simulink model "pfb_fft_d3a"  (R2021a)
settings: Solver=VariableStepAuto  StartTime=0.0  StopTime=100.0  RelTol=1e-3
undefined symbols (not defined in the file): i, pfb_coeff_gen_calc
libraries: xbsIndex_r4 x11529, casper_library_misc x39, casper_library_delays x39, xbsReplacements_r4 x2
(part 38 of 118)

== system pfb_fft_d3a/fft_wideband_real/fft_biplex_real_4x/bi_real_unscr_4x/mirror_spectrum/dmux2 ==
  sel : Inport
  d0 : Inport  Port=2
  d1 : Inport  Port=3
  d_bussify : Subsystem  AncestorBlock=casper_library_flow_control/bus_create  mask(bus_create){inputNum=2}
      mask prompts: inputNum "Number of inputs:"
      mask init:
      | bus_create_init(gcb,...
      |     'inputNum', inputNum);
  expand0 : Subsystem  AncestorBlock=casper_library_flow_control/bus_expand  mask(bus_expand){mode=divisions of arbitrary size, outputNum=2, outputWidth=[36 36], outputBinaryPt=[0  0], outputArithmeticType=[0  0], show_format=on, outputToWorkspace=off, variablePrefix=, outputToModelAsWell=on}
      mask prompts: outputNum "Number of outputs:"; outputWidth "Output width:"; outputBinaryPt "Output binary point position:"; outputArithmeticType "Output arithmetic type (ufix=0, fix=1, bool=2):"; show_format "Print format string?"; outputToWorkspace "Output to workspace?"; variablePrefix "Variable name prefix:"; outputToModelAsWell "Output to model as well?"
      mask help:
      | Expands a 'bus' made using a bus_create or Xilinx
      | concat block.
      | The input will be divided into the specified number
      | of outputs with the specified arithmetic types.
      | Divisions are made from most significant bit.
      mask init: same as pfb_fft_d3a/fft_wideband_real/fft_biplex_real_4x/pol0_debus
      settings: AttributesFormatString=2 outputs: uf36.0,uf36.0,
      mask TypeOptions mode: divisions of equal size | divisions of arbitrary size
      mask Callback mode: %bus_expand_callback();
      mask Callback outputWidth: %bus_expand_callback();
      mask Callback outputToWorkspace: %bus_expand_callback();
  expand1 : Subsystem  AncestorBlock=casper_library_flow_control/bus_expand  mask(bus_expand){mode=divisions of arbitrary size, outputNum=2, outputWidth=[36 36], outputBinaryPt=[0  0], outputArithmeticType=[0  0], show_format=on, outputToWorkspace=off, variablePrefix=, outputToModelAsWell=on}
      mask prompts: outputNum "Number of outputs:"; outputWidth "Output width:"; outputBinaryPt "Output binary point position:"; outputArithmeticType "Output arithmetic type (ufix=0, fix=1, bool=2):"; show_format "Print format string?"; outputToWorkspace "Output to workspace?"; variablePrefix "Variable name prefix:"; outputToModelAsWell "Output to model as well?"
      mask help:
      | Expands a 'bus' made using a bus_create or Xilinx
      | concat block.
      | The input will be divided into the specified number
      | of outputs with the specified arithmetic types.
      | Divisions are made from most significant bit.
      mask init: same as pfb_fft_d3a/fft_wideband_real/fft_biplex_real_4x/pol0_debus
      settings: AttributesFormatString=2 outputs: uf36.0,uf36.0,
      mask TypeOptions mode: divisions of equal size | divisions of arbitrary size
      mask Callback mode: %bus_expand_callback();
      mask Callback outputWidth: %bus_expand_callback();
      mask Callback outputToWorkspace: %bus_expand_callback();
  mux0 : xbsIndex_r4/Mux  inputs=2  en=off  latency=1  precision=Full  arith_type=Unsigned  n_bits=16  bin_pt=14  quantization=Truncate  overflow=Wrap  dbl_ovrd=off  block_type=mux
  mux1 : xbsIndex_r4/Mux  inputs=2  en=off  latency=1  precision=Full  arith_type=Unsigned  n_bits=16  bin_pt=14  quantization=Truncate  overflow=Wrap  dbl_ovrd=off  block_type=mux
  sel_expand : Subsystem  AncestorBlock=casper_library_flow_control/bus_expand  mask(bus_expand){mode=divisions of equal size, outputNum=2, outputWidth=1, outputBinaryPt=0, outputArithmeticType=0, show_format=on, outputToWorkspace=off, variablePrefix=, outputToModelAsWell=on}
      mask prompts: outputNum "Number of outputs:"; outputWidth "Output width:"; outputBinaryPt "Output binary point position:"; outputArithmeticType "Output arithmetic type (ufix=0, fix=1, bool=2):"; show_format "Print format string?"; outputToWorkspace "Output to workspace?"; variablePrefix "Variable name prefix:"; outputToModelAsWell "Output to model as well?"
      mask help:
      | Expands a 'bus' made using a bus_create or Xilinx
      | concat block.
      | The input will be divided into the specified number
      | of outputs with the specified arithmetic types.
      | Divisions are made from most significant bit.
      mask init: same as pfb_fft_d3a/fft_wideband_real/fft_biplex_real_4x/pol0_debus
      settings: AttributesFormatString=2 outputs: uf1.0,uf1.0,
      mask TypeOptions mode: divisions of equal size | divisions of arbitrary size
      mask Callback mode: %bus_expand_callback();
      mask Callback outputWidth: %bus_expand_callback();
      mask Callback outputToWorkspace: %bus_expand_callback();
  out : Outport
  wires:
  sel/1 -> sel_expand/1(bus_in)
  d0/1 -> expand0/1(bus_in)
  d1/1 -> expand1/1(bus_in)
  sel_expand/1(msb_out2) -> mux0/1
  expand0/1(msb_out2) -> mux0/2
  expand1/1(msb_out2) -> mux0/3
  sel_expand/2(lsb_out1) -> mux1/1
  expand0/2(lsb_out1) -> mux1/2
  expand1/2(lsb_out1) -> mux1/3
  mux0/1 -> d_bussify/1(in1)
  mux1/1 -> d_bussify/2(in2)
  d_bussify/1(bus_out) -> out/1

== system pfb_fft_d3a/fft_wideband_real/fft_biplex_real_4x/bi_real_unscr_4x/mirror_spectrum/dmux3 ==
  sel : Inport
  d0 : Inport  Port=2
  d1 : Inport  Port=3
  d_bussify : Subsystem  AncestorBlock=casper_library_flow_control/bus_create  mask(bus_create){inputNum=2}
      mask prompts: inputNum "Number of inputs:"
      mask init:
      | bus_create_init(gcb,...
      |     'inputNum', inputNum);
  expand0 : Subsystem  AncestorBlock=casper_library_flow_control/bus_expand  mask(bus_expand){mode=divisions of arbitrary size, outputNum=2, outputWidth=[36 36], outputBinaryPt=[0  0], outputArithmeticType=[0  0], show_format=on, outputToWorkspace=off, variablePrefix=, outputToModelAsWell=on}
      mask prompts: outputNum "Number of outputs:"; outputWidth "Output width:"; outputBinaryPt "Output binary point position:"; outputArithmeticType "Output arithmetic type (ufix=0, fix=1, bool=2):"; show_format "Print format string?"; outputToWorkspace "Output to workspace?"; variablePrefix "Variable name prefix:"; outputToModelAsWell "Output to model as well?"
      mask help:
      | Expands a 'bus' made using a bus_create or Xilinx
      | concat block.
      | The input will be divided into the specified number
      | of outputs with the specified arithmetic types.
      | Divisions are made from most significant bit.
      mask init: same as pfb_fft_d3a/fft_wideband_real/fft_biplex_real_4x/pol0_debus
      settings: AttributesFormatString=2 outputs: uf36.0,uf36.0,
      mask TypeOptions mode: divisions of equal size | divisions of arbitrary size
      mask Callback mode: %bus_expand_callback();
      mask Callback outputWidth: %bus_expand_callback();
      mask Callback outputToWorkspace: %bus_expand_callback();
  expand1 : Subsystem  AncestorBlock=casper_library_flow_control/bus_expand  mask(bus_expand){mode=divisions of arbitrary size, outputNum=2, outputWidth=[36 36], outputBinaryPt=[0  0], outputArithmeticType=[0  0], show_format=on, outputToWorkspace=off, variablePrefix=, outputToModelAsWell=on}
      mask prompts: outputNum "Number of outputs:"; outputWidth "Output width:"; outputBinaryPt "Output binary point position:"; outputArithmeticType "Output arithmetic type (ufix=0, fix=1, bool=2):"; show_format "Print format string?"; outputToWorkspace "Output to workspace?"; variablePrefix "Variable name prefix:"; outputToModelAsWell "Output to model as well?"
      mask help:
      | Expands a 'bus' made using a bus_create or Xilinx
      | concat block.
      | The input will be divided into the specified number
      | of outputs with the specified arithmetic types.
      | Divisions are made from most significant bit.
      mask init: same as pfb_fft_d3a/fft_wideband_real/fft_biplex_real_4x/pol0_debus
      settings: AttributesFormatString=2 outputs: uf36.0,uf36.0,
      mask TypeOptions mode: divisions of equal size | divisions of arbitrary size
      mask Callback mode: %bus_expand_callback();
      mask Callback outputWidth: %bus_expand_callback();
      mask Callback outputToWorkspace: %bus_expand_callback();
  mux0 : xbsIndex_r4/Mux  inputs=2  en=off  latency=1  precision=Full  arith_type=Unsigned  n_bits=16  bin_pt=14  quantization=Truncate  overflow=Wrap  dbl_ovrd=off  block_type=mux
  mux1 : xbsIndex_r4/Mux  inputs=2  en=off  latency=1  precision=Full  arith_type=Unsigned  n_bits=16  bin_pt=14  quantization=Truncate  overflow=Wrap  dbl_ovrd=off  block_type=mux
  sel_expand : Subsystem  AncestorBlock=casper_library_flow_control/bus_expand  mask(bus_expand){mode=divisions of equal size, outputNum=2, outputWidth=1, outputBinaryPt=0, outputArithmeticType=0, show_format=on, outputToWorkspace=off, variablePrefix=, outputToModelAsWell=on}
      mask prompts: outputNum "Number of outputs:"; outputWidth "Output width:"; outputBinaryPt "Output binary point position:"; outputArithmeticType "Output arithmetic type (ufix=0, fix=1, bool=2):"; show_format "Print format string?"; outputToWorkspace "Output to workspace?"; variablePrefix "Variable name prefix:"; outputToModelAsWell "Output to model as well?"
      mask help:
      | Expands a 'bus' made using a bus_create or Xilinx
      | concat block.
      | The input will be divided into the specified number
      | of outputs with the specified arithmetic types.
      | Divisions are made from most significant bit.
      mask init: same as pfb_fft_d3a/fft_wideband_real/fft_biplex_real_4x/pol0_debus
      settings: AttributesFormatString=2 outputs: uf1.0,uf1.0,
      mask TypeOptions mode: divisions of equal size | divisions of arbitrary size
      mask Callback mode: %bus_expand_callback();
      mask Callback outputWidth: %bus_expand_callback();
      mask Callback outputToWorkspace: %bus_expand_callback();
  out : Outport
  wires:
  sel/1 -> sel_expand/1(bus_in)
  d0/1 -> expand0/1(bus_in)
  d1/1 -> expand1/1(bus_in)
  sel_expand/1(msb_out2) -> mux0/1
  expand0/1(msb_out2) -> mux0/2
  expand1/1(msb_out2) -> mux0/3
  sel_expand/2(lsb_out1) -> mux1/1
  expand0/2(lsb_out1) -> mux1/2
  expand1/2(lsb_out1) -> mux1/3
  mux0/1 -> d_bussify/1(in1)
  mux1/1 -> d_bussify/2(in2)
  d_bussify/1(bus_out) -> out/1

== system pfb_fft_d3a/fft_wideband_real/fft_biplex_real_4x/bi_real_unscr_4x/mirror_spectrum/sel_replicate0 ==
  in : Inport
  bussify : Subsystem  AncestorBlock=casper_library_flow_control/bus_create  mask(bus_create){inputNum=2}
      mask prompts: inputNum "Number of inputs:"
      mask init:
      | bus_create_init(gcb,...
      |     'inputNum', inputNum);
  din0_0 : xbsIndex_r4/Delay  rst=off  infoeditControl=Selection of Reset will increase slice count due to use of real FFs and instead of SRLs  en=off  latency=1  reg_retiming=off  dbl_ovrd=off  block_type=delay
  din0_1 : xbsIndex_r4/Delay  rst=off  infoeditControl=Selection of Reset will increase slice count due to use of real FFs and instead of SRLs  en=off  latency=1  reg_retiming=off  dbl_ovrd=off  block_type=delay
  out : Outport
  wires:
  in/1 -> din0_0/1, din0_1/1
  din0_0/1 -> bussify/1(in1)
  din0_1/1 -> bussify/2(in2)
  bussify/1(bus_out) -> out/1

== system pfb_fft_d3a/fft_wideband_real/fft_biplex_real_4x/bi_real_unscr_4x/mirror_spectrum/sel_replicate1 ==
  in : Inport
  bussify : Subsystem  AncestorBlock=casper_library_flow_control/bus_create  mask(bus_create){inputNum=2}
      mask prompts: inputNum "Number of inputs:"
      mask init:
      | bus_create_init(gcb,...
      |     'inputNum', inputNum);
  din0_0 : xbsIndex_r4/Delay  rst=off  infoeditControl=Selection of Reset will increase slice count due to use of real FFs and instead of SRLs  en=off  latency=1  reg_retiming=off  dbl_ovrd=off  block_type=delay
  din0_1 : xbsIndex_r4/Delay  rst=off  infoeditControl=Selection of Reset will increase slice count due to use of real FFs and instead of SRLs  en=off  latency=1  reg_retiming=off  dbl_ovrd=off  block_type=delay
  out : Outport
  wires:
  in/1 -> din0_0/1, din0_1/1
  din0_0/1 -> bussify/1(in1)
  din0_1/1 -> bussify/2(in2)
  bussify/1(bus_out) -> out/1

== system pfb_fft_d3a/fft_wideband_real/fft_biplex_real_4x/bi_real_unscr_4x/mirror_spectrum/sel_replicate2 ==
  in : Inport
  bussify : Subsystem  AncestorBlock=casper_library_flow_control/bus_create  mask(bus_create){inputNum=2}
      mask prompts: inputNum "Number of inputs:"
      mask init:
      | bus_create_init(gcb,...
      |     'inputNum', inputNum);
  din0_0 : xbsIndex_r4/Delay  rst=off  infoeditControl=Selection of Reset will increase slice count due to use of real FFs and instead of SRLs  en=off  latency=1  reg_retiming=off  dbl_ovrd=off  block_type=delay
  din0_1 : xbsIndex_r4/Delay  rst=off  infoeditControl=Selection of Reset will increase slice count due to use of real FFs and instead of SRLs  en=off  latency=1  reg_retiming=off  dbl_ovrd=off  block_type=delay
  out : Outport
  wires:
  in/1 -> din0_0/1, din0_1/1
  din0_0/1 -> bussify/1(in1)
  din0_1/1 -> bussify/2(in2)
  bussify/1(bus_out) -> out/1

== system pfb_fft_d3a/fft_wideband_real/fft_biplex_real_4x/bi_real_unscr_4x/mirror_spectrum/sel_replicate3 ==
  in : Inport
  bussify : Subsystem  AncestorBlock=casper_library_flow_control/bus_create  mask(bus_create){inputNum=2}
      mask prompts: inputNum "Number of inputs:"
      mask init:
      | bus_create_init(gcb,...
      |     'inputNum', inputNum);
  din0_0 : xbsIndex_r4/Delay  rst=off  infoeditControl=Selection of Reset will increase slice count due to use of real FFs and instead of SRLs  en=off  latency=1  reg_retiming=off  dbl_ovrd=off  block_type=delay
  din0_1 : xbsIndex_r4/Delay  rst=off  infoeditControl=Selection of Reset will increase slice count due to use of real FFs and instead of SRLs  en=off  latency=1  reg_retiming=off  dbl_ovrd=off  block_type=delay
  out : Outport
  wires:
  in/1 -> din0_0/1, din0_1/1
  din0_0/1 -> bussify/1(in1)
  din0_1/1 -> bussify/2(in2)
  bussify/1(bus_out) -> out/1

== system pfb_fft_d3a/fft_wideband_real/fft_biplex_real_4x/bi_real_unscr_4x/reorder_even/addr_expand ==
  bus_in : Inport
  reinterpret1 : xbsIndex_r4/Reinterpret  force_arith_type=on  arith_type=Unsigned  force_bin_pt=on  bin_pt=0  block_type=reinterpret
  slice1 : xbsIndex_r4/Slice  nbits=10  boolean_output=off  mode=Upper Bit Location + Width  bit1=0  base1=MSB of Input  bit0=0  base0=LSB of Input  dbl_ovrd=off  block_type=slice
  msb_lsb_out1 : Outport
  wires:
  bus_in/1 -> slice1/1
  slice1/1 -> reinterpret1/1
  reinterpret1/1 -> msb_lsb_out1/1

== system pfb_fft_d3a/fft_wideband_real/fft_biplex_real_4x/bi_real_unscr_4x/reorder_even/addr_replicate ==
  in : Inport
  bussify : Subsystem  AncestorBlock=casper_library_flow_control/bus_create  mask(bus_create){inputNum=1}
      mask prompts: inputNum "Number of inputs:"
      mask init:
      | bus_create_init(gcb,...
      |     'inputNum', inputNum);
  out : Outport
  wires:
  in/1 -> bussify/1(in1)
  bussify/1(bus_out) -> out/1

== system pfb_fft_d3a/fft_wideband_real/fft_biplex_real_4x/bi_real_unscr_4x/reorder_even/buf0 ==
  addr : Inport
  din : Inport  Port=2
  we : Inport  Port=3
  bram{0..3} (4 alike) : xbsIndex_r4/Single Port RAM  depth=1024  initVector=getfield(get_param(gcb, 'UserData'), 'initVector')  distributed_mem=Block RAM  write_mode=Read Before Write  rst=off  init_reg=0  en=off  optimize_latency=off  latency=2  optimize=Speed  dbl_ovrd=off  simulation_type=fast_sim  block_type=spram
  ddin : xbsIndex_r4/Delay  rst=off  infoeditControl=Selection of Reset will increase slice count due to use of real FFs and instead of SRLs  en=off  latency=3  reg_retiming=on  dbl_ovrd=off  block_type=delay
  debus_addr : Subsystem  AncestorBlock=casper_library_flow_control/bus_expand  mask(bus_expand){mode=divisions of equal size, outputNum=4, outputWidth=[10 10 10 10], outputBinaryPt=[0 0 0 0], outputArithmeticType=[0 0 0 0], show_format=on, outputToWorkspace=off, variablePrefix=, outputToModelAsWell=on}
      mask prompts: outputNum "Number of outputs:"; outputWidth "Output width:"; outputBinaryPt "Output binary point position:"; outputArithmeticType "Output arithmetic type (ufix=0, fix=1, bool=2):"; show_format "Print format string?"; outputToWorkspace "Output to workspace?"; variablePrefix "Variable name prefix:"; outputToModelAsWell "Output to model as well?"
      mask help:
      | Expands a 'bus' made using a bus_create or Xilinx
      | concat block.
      | The input will be divided into the specified number
      | of outputs with the specified arithmetic types.
      | Divisions are made from most significant bit.
      mask init: same as pfb_fft_d3a/fft_wideband_real/fft_biplex_real_4x/pol0_debus
      settings: AttributesFormatString=4 outputs: uf10.0,uf10.0,uf10.0,uf10.0,
      mask TypeOptions mode: divisions of equal size | divisions of arbitrary size
      mask Callback mode: %bus_expand_callback();
      mask Callback outputWidth: %bus_expand_callback();
      mask Callback outputToWorkspace: %bus_expand_callback();
  debus_din : Subsystem  AncestorBlock=casper_library_flow_control/bus_expand  mask(bus_expand){mode=divisions of arbitrary size, outputNum=2, outputWidth=[18 18 18 18], outputBinaryPt=[0 0 0 0], outputArithmeticType=[0 0 0 0], show_format=on, outputToWorkspace=off, variablePrefix=, outputToModelAsWell=on}
      mask prompts: outputNum "Number of outputs:"; outputWidth "Output width:"; outputBinaryPt "Output binary point position:"; outputArithmeticType "Output arithmetic type (ufix=0, fix=1, bool=2):"; show_format "Print format string?"; outputToWorkspace "Output to workspace?"; variablePrefix "Variable name prefix:"; outputToModelAsWell "Output to model as well?"
      mask help:
      | Expands a 'bus' made using a bus_create or Xilinx
      | concat block.
      | The input will be divided into the specified number
      | of outputs with the specified arithmetic types.
      | Divisions are made from most significant bit.
      mask init: same as pfb_fft_d3a/fft_wideband_real/fft_biplex_real_4x/pol0_debus
      settings: AttributesFormatString=4 outputs: uf18.0,uf18.0,uf18.0,uf18.0,
      mask TypeOptions mode: divisions of equal size | divisions of arbitrary size
      mask Callback mode: %bus_expand_callback();
      mask Callback outputWidth: %bus_expand_callback();
      mask Callback outputToWorkspace: %bus_expand_callback();
  debus_we : Subsystem  AncestorBlock=casper_library_flow_control/bus_expand  mask(bus_expand){mode=divisions of equal size, outputNum=4, outputWidth=[1 1 1 1], outputBinaryPt=[0 0 0 0], outputArithmeticType=[2 2 2 2], show_format=on, outputToWorkspace=off, variablePrefix=, outputToModelAsWell=on}
      mask prompts: outputNum "Number of outputs:"; outputWidth "Output width:"; outputBinaryPt "Output binary point position:"; outputArithmeticType "Output arithmetic type (ufix=0, fix=1, bool=2):"; show_format "Print format string?"; outputToWorkspace "Output to workspace?"; variablePrefix "Variable name prefix:"; outputToModelAsWell "Output to model as well?"
      mask help:
      | Expands a 'bus' made using a bus_create or Xilinx
      | concat block.
      | The input will be divided into the specified number
      | of outputs with the specified arithmetic types.
      | Divisions are made from most significant bit.
      mask init: same as pfb_fft_d3a/fft_wideband_real/fft_biplex_real_4x/pol0_debus
      settings: AttributesFormatString=4 outputs: b,b,b,b,
      mask TypeOptions mode: divisions of equal size | divisions of arbitrary size
      mask Callback mode: %bus_expand_callback();
      mask Callback outputWidth: %bus_expand_callback();
      mask Callback outputToWorkspace: %bus_expand_callback();
  din_bussify : Subsystem  AncestorBlock=casper_library_flow_control/bus_create  mask(bus_create){inputNum=4}
      mask prompts: inputNum "Number of inputs:"
      mask init:
      | bus_create_init(gcb,...
      |     'inputNum', inputNum);
  rep_addr : Subsystem  AncestorBlock=casper_library_bus/bus_replicate  mask(bus_replicate){replication=4, csp_latency=3, misc=off, implementation=core}
      mask prompts: replication "replication factor"; csp_latency "latency"; misc "misc support"; implementation "delay implementation"
      mask help: Output bus formed by replicating input bus a number of times
      mask init:
      | bus_replicate_init(gcb, ...
      |     'replication', replication, ...
      |     'csp_latency', csp_latency, ...
      |     'implementation', implementation, ...
      |     'misc', misc);
      mask TypeOptions implementation: core | behavioral
  rep_we : Subsystem  AncestorBlock=casper_library_bus/bus_replicate  mask(bus_replicate){replication=4, csp_latency=3, misc=off, implementation=core}
      mask prompts: replication "replication factor"; csp_latency "latency"; misc "misc support"; implementation "delay implementation"
      mask help: Output bus formed by replicating input bus a number of times
      mask init:
      | bus_replicate_init(gcb, ...
      |     'replication', replication, ...
      |     'csp_latency', csp_latency, ...
      |     'implementation', implementation, ...
      |     'misc', misc);
      mask TypeOptions implementation: core | behavioral
  dout : Outport
  wires:
  addr/1 -> rep_addr/1(in)
  din/1 -> ddin/1
  we/1 -> rep_we/1(in)
  rep_addr/1(out) -> debus_addr/1(bus_in)
  ddin/1 -> debus_din/1(bus_in)
  rep_we/1(out) -> debus_we/1(bus_in)
  debus_addr/1(msb_out4) -> bram0/1
  debus_din/1(msb_out4) -> bram0/2
  debus_we/1(msb_out4) -> bram0/3
  debus_addr/2(out3) -> bram1/1
  debus_din/2(out3) -> bram1/2
  debus_we/2(out3) -> bram1/3
  debus_addr/3(out2) -> bram2/1
  debus_din/3(out2) -> bram2/2
  debus_we/3(out2) -> bram2/3
  debus_addr/4(lsb_out1) -> bram3/1
  debus_din/4(lsb_out1) -> bram3/2
  debus_we/4(lsb_out1) -> bram3/3
  bram0/1 -> din_bussify/1(in1)
  bram1/1 -> din_bussify/2(in2)
  bram2/1 -> din_bussify/3(in3)
  bram3/1 -> din_bussify/4(in4)
  din_bussify/1(bus_out) -> dout/1

== system pfb_fft_d3a/fft_wideband_real/fft_biplex_real_4x/bi_real_unscr_4x/reorder_even/we_expand ==
  bus_in : Inport
  slice1 : xbsIndex_r4/Slice  nbits=1  boolean_output=on  mode=Upper Bit Location + Width  bit1=0  base1=MSB of Input  bit0=0  base0=LSB of Input  dbl_ovrd=off  block_type=slice
  msb_lsb_out1 : Outport
  wires:
  bus_in/1 -> slice1/1
  slice1/1 -> msb_lsb_out1/1

== system pfb_fft_d3a/fft_wideband_real/fft_biplex_real_4x/bi_real_unscr_4x/reorder_even/we_replicate ==
  in : Inport
  bussify : Subsystem  AncestorBlock=casper_library_flow_control/bus_create  mask(bus_create){inputNum=1}
      mask prompts: inputNum "Number of inputs:"
      mask init:
      | bus_create_init(gcb,...
      |     'inputNum', inputNum);
  out : Outport
  wires:
  in/1 -> bussify/1(in1)
  bussify/1(bus_out) -> out/1

== system pfb_fft_d3a/fft_wideband_real/fft_biplex_real_4x/bi_real_unscr_4x/reorder_odd/addr_expand ==
  bus_in : Inport
  reinterpret1 : xbsIndex_r4/Reinterpret  force_arith_type=on  arith_type=Unsigned  force_bin_pt=on  bin_pt=0  block_type=reinterpret
  slice1 : xbsIndex_r4/Slice  nbits=10  boolean_output=off  mode=Upper Bit Location + Width  bit1=0  base1=MSB of Input  bit0=0  base0=LSB of Input  dbl_ovrd=off  block_type=slice
  msb_lsb_out1 : Outport
  wires:
  bus_in/1 -> slice1/1
  slice1/1 -> reinterpret1/1
  reinterpret1/1 -> msb_lsb_out1/1

== system pfb_fft_d3a/fft_wideband_real/fft_biplex_real_4x/bi_real_unscr_4x/reorder_odd/addr_replicate ==
  in : Inport
  bussify : Subsystem  AncestorBlock=casper_library_flow_control/bus_create  mask(bus_create){inputNum=1}
      mask prompts: inputNum "Number of inputs:"
      mask init:
      | bus_create_init(gcb,...
      |     'inputNum', inputNum);
  out : Outport
  wires:
  in/1 -> bussify/1(in1)
  bussify/1(bus_out) -> out/1

== system pfb_fft_d3a/fft_wideband_real/fft_biplex_real_4x/bi_real_unscr_4x/reorder_odd/buf0 ==
  addr : Inport
  din : Inport  Port=2
  we : Inport  Port=3
  bram{0..3} (4 alike) : xbsIndex_r4/Single Port RAM  depth=1024  initVector=getfield(get_param(gcb, 'UserData'), 'initVector')  distributed_mem=Block RAM  write_mode=Read Before Write  rst=off  init_reg=0  en=off  optimize_latency=off  latency=2  optimize=Speed  dbl_ovrd=off  simulation_type=fast_sim  block_type=spram
  ddin : xbsIndex_r4/Delay  rst=off  infoeditControl=Selection of Reset will increase slice count due to use of real FFs and instead of SRLs  en=off  latency=3  reg_retiming=on  dbl_ovrd=off  block_type=delay
  debus_addr : Subsystem  AncestorBlock=casper_library_flow_control/bus_expand  mask(bus_expand){mode=divisions of equal size, outputNum=4, outputWidth=[10 10 10 10], outputBinaryPt=[0 0 0 0], outputArithmeticType=[0 0 0 0], show_format=on, outputToWorkspace=off, variablePrefix=, outputToModelAsWell=on}
      mask prompts: outputNum "Number of outputs:"; outputWidth "Output width:"; outputBinaryPt "Output binary point position:"; outputArithmeticType "Output arithmetic type (ufix=0, fix=1, bool=2):"; show_format "Print format string?"; outputToWorkspace "Output to workspace?"; variablePrefix "Variable name prefix:"; outputToModelAsWell "Output to model as well?"
      mask help:
      | Expands a 'bus' made using a bus_create or Xilinx
      | concat block.
      | The input will be divided into the specified number
      | of outputs with the specified arithmetic types.
      | Divisions are made from most significant bit.
      mask init: same as pfb_fft_d3a/fft_wideband_real/fft_biplex_real_4x/pol0_debus
      settings: AttributesFormatString=4 outputs: uf10.0,uf10.0,uf10.0,uf10.0,
      mask TypeOptions mode: divisions of equal size | divisions of arbitrary size
      mask Callback mode: %bus_expand_callback();
      mask Callback outputWidth: %bus_expand_callback();
      mask Callback outputToWorkspace: %bus_expand_callback();
  debus_din : Subsystem  AncestorBlock=casper_library_flow_control/bus_expand  mask(bus_expand){mode=divisions of arbitrary size, outputNum=2, outputWidth=[18 18 18 18], outputBinaryPt=[0 0 0 0], outputArithmeticType=[0 0 0 0], show_format=on, outputToWorkspace=off, variablePrefix=, outputToModelAsWell=on}
      mask prompts: outputNum "Number of outputs:"; outputWidth "Output width:"; outputBinaryPt "Output binary point position:"; outputArithmeticType "Output arithmetic type (ufix=0, fix=1, bool=2):"; show_format "Print format string?"; outputToWorkspace "Output to workspace?"; variablePrefix "Variable name prefix:"; outputToModelAsWell "Output to model as well?"
      mask help:
      | Expands a 'bus' made using a bus_create or Xilinx
      | concat block.
      | The input will be divided into the specified number
      | of outputs with the specified arithmetic types.
      | Divisions are made from most significant bit.
      mask init: same as pfb_fft_d3a/fft_wideband_real/fft_biplex_real_4x/pol0_debus
      settings: AttributesFormatString=4 outputs: uf18.0,uf18.0,uf18.0,uf18.0,
      mask TypeOptions mode: divisions of equal size | divisions of arbitrary size
      mask Callback mode: %bus_expand_callback();
      mask Callback outputWidth: %bus_expand_callback();
      mask Callback outputToWorkspace: %bus_expand_callback();
  debus_we : Subsystem  AncestorBlock=casper_library_flow_control/bus_expand  mask(bus_expand){mode=divisions of equal size, outputNum=4, outputWidth=[1 1 1 1], outputBinaryPt=[0 0 0 0], outputArithmeticType=[2 2 2 2], show_format=on, outputToWorkspace=off, variablePrefix=, outputToModelAsWell=on}
      mask prompts: outputNum "Number of outputs:"; outputWidth "Output width:"; outputBinaryPt "Output binary point position:"; outputArithmeticType "Output arithmetic type (ufix=0, fix=1, bool=2):"; show_format "Print format string?"; outputToWorkspace "Output to workspace?"; variablePrefix "Variable name prefix:"; outputToModelAsWell "Output to model as well?"
      mask help:
      | Expands a 'bus' made using a bus_create or Xilinx
      | concat block.
      | The input will be divided into the specified number
      | of outputs with the specified arithmetic types.
      | Divisions are made from most significant bit.
      mask init: same as pfb_fft_d3a/fft_wideband_real/fft_biplex_real_4x/pol0_debus
      settings: AttributesFormatString=4 outputs: b,b,b,b,
      mask TypeOptions mode: divisions of equal size | divisions of arbitrary size
      mask Callback mode: %bus_expand_callback();
      mask Callback outputWidth: %bus_expand_callback();
      mask Callback outputToWorkspace: %bus_expand_callback();
  din_bussify : Subsystem  AncestorBlock=casper_library_flow_control/bus_create  mask(bus_create){inputNum=4}
      mask prompts: inputNum "Number of inputs:"
      mask init:
      | bus_create_init(gcb,...
      |     'inputNum', inputNum);
  rep_addr : Subsystem  AncestorBlock=casper_library_bus/bus_replicate  mask(bus_replicate){replication=4, csp_latency=3, misc=off, implementation=core}
      mask prompts: replication "replication factor"; csp_latency "latency"; misc "misc support"; implementation "delay implementation"
      mask help: Output bus formed by replicating input bus a number of times
      mask init:
      | bus_replicate_init(gcb, ...
      |     'replication', replication, ...
      |     'csp_latency', csp_latency, ...
      |     'implementation', implementation, ...
      |     'misc', misc);
      mask TypeOptions implementation: core | behavioral
  rep_we : Subsystem  AncestorBlock=casper_library_bus/bus_replicate  mask(bus_replicate){replication=4, csp_latency=3, misc=off, implementation=core}
      mask prompts: replication "replication factor"; csp_latency "latency"; misc "misc support"; implementation "delay implementation"
      mask help: Output bus formed by replicating input bus a number of times
      mask init:
      | bus_replicate_init(gcb, ...
      |     'replication', replication, ...
      |     'csp_latency', csp_latency, ...
      |     'implementation', implementation, ...
      |     'misc', misc);
      mask TypeOptions implementation: core | behavioral
  dout : Outport
  wires:
  addr/1 -> rep_addr/1(in)
  din/1 -> ddin/1
  we/1 -> rep_we/1(in)
  rep_addr/1(out) -> debus_addr/1(bus_in)
  ddin/1 -> debus_din/1(bus_in)
  rep_we/1(out) -> debus_we/1(bus_in)
  debus_addr/1(msb_out4) -> bram0/1
  debus_din/1(msb_out4) -> bram0/2
  debus_we/1(msb_out4) -> bram0/3
  debus_addr/2(out3) -> bram1/1
  debus_din/2(out3) -> bram1/2
  debus_we/2(out3) -> bram1/3
  debus_addr/3(out2) -> bram2/1
  debus_din/3(out2) -> bram2/2
  debus_we/3(out2) -> bram2/3
  debus_addr/4(lsb_out1) -> bram3/1
  debus_din/4(lsb_out1) -> bram3/2
  debus_we/4(lsb_out1) -> bram3/3
  bram0/1 -> din_bussify/1(in1)
  bram1/1 -> din_bussify/2(in2)
  bram2/1 -> din_bussify/3(in3)
  bram3/1 -> din_bussify/4(in4)
  din_bussify/1(bus_out) -> dout/1

== system pfb_fft_d3a/fft_wideband_real/fft_biplex_real_4x/bi_real_unscr_4x/reorder_odd/we_expand ==
  bus_in : Inport
  slice1 : xbsIndex_r4/Slice  nbits=1  boolean_output=on  mode=Upper Bit Location + Width  bit1=0  base1=MSB of Input  bit0=0  base0=LSB of Input  dbl_ovrd=off  block_type=slice
  msb_lsb_out1 : Outport
  wires:
  bus_in/1 -> slice1/1
  slice1/1 -> msb_lsb_out1/1

== system pfb_fft_d3a/fft_wideband_real/fft_biplex_real_4x/bi_real_unscr_4x/reorder_odd/we_replicate ==
  in : Inport
  bussify : Subsystem  AncestorBlock=casper_library_flow_control/bus_create  mask(bus_create){inputNum=1}
      mask prompts: inputNum "Number of inputs:"
      mask init:
      | bus_create_init(gcb,...
      |     'inputNum', inputNum);
  out : Outport
  wires:
  in/1 -> bussify/1(in1)
  bussify/1(bus_out) -> out/1

== system pfb_fft_d3a/fft_wideband_real/fft_biplex_real_4x/bi_real_unscr_4x/reorder_out/addr_expand ==
  bus_in : Inport
  reinterpret{1..4} (4 alike) : xbsIndex_r4/Reinterpret  force_arith_type=on  arith_type=Unsigned  force_bin_pt=on  bin_pt=0  block_type=reinterpret
  slice1 : xbsIndex_r4/Slice  nbits=10  boolean_output=off  mode=Upper Bit Location + Width  bit1=-30  base1=MSB of Input  bit0=0  base0=LSB of Input  dbl_ovrd=off  block_type=slice
  slice2 : xbsIndex_r4/Slice  nbits=10  boolean_output=off  mode=Upper Bit Location + Width  bit1=-20  base1=MSB of Input  bit0=0  base0=LSB of Input  dbl_ovrd=off  block_type=slice
  slice3 : xbsIndex_r4/Slice  nbits=10  boolean_output=off  mode=Upper Bit Location + Width  bit1=-10  base1=MSB of Input  bit0=0  base0=LSB of Input  dbl_ovrd=off  block_type=slice
  slice4 : xbsIndex_r4/Slice  nbits=10  boolean_output=off  mode=Upper Bit Location + Width  bit1=0  base1=MSB of Input  bit0=0  base0=LSB of Input  dbl_ovrd=off  block_type=slice
  msb_out4 : Outport
  out3 : Outport  Port=2
  out2 : Outport  Port=3
  lsb_out1 : Outport  Port=4  VectorParamsAs1DForOutWhenUnconnected=off
  wires:
  bus_in/1 -> slice4/1, slice3/1, slice2/1, slice1/1
  slice4/1 -> reinterpret4/1
  reinterpret4/1 -> msb_out4/1
  slice3/1 -> reinterpret3/1
  reinterpret3/1 -> out3/1
  slice2/1 -> reinterpret2/1
  reinterpret2/1 -> out2/1
  slice1/1 -> reinterpret1/1
  reinterpret1/1 -> lsb_out1/1

== system pfb_fft_d3a/fft_wideband_real/fft_biplex_real_4x/bi_real_unscr_4x/reorder_out/addr_replicate ==
  in : Inport
  bussify : Subsystem  AncestorBlock=casper_library_flow_control/bus_create  mask(bus_create){inputNum=4}
      mask prompts: inputNum "Number of inputs:"
      mask init:
      | bus_create_init(gcb,...
      |     'inputNum', inputNum);
  din0_0 : xbsIndex_r4/Delay  rst=off  infoeditControl=Selection of Reset will increase slice count due to use of real FFs and instead of SRLs  en=off  latency=1  reg_retiming=off  dbl_ovrd=off  block_type=delay
  din0_1 : xbsIndex_r4/Delay  rst=off  infoeditControl=Selection of Reset will increase slice count due to use of real FFs and instead of SRLs  en=off  latency=1  reg_retiming=off  dbl_ovrd=off  block_type=delay
  din1_{0..3} (4 alike) : xbsIndex_r4/Delay  rst=off  infoeditControl=Selection of Reset will increase slice count due to use of real FFs and instead of SRLs  en=off  latency=1  reg_retiming=off  dbl_ovrd=off  block_type=delay
  out : Outport
  wires:
  in/1 -> din0_0/1, din0_1/1
  din0_0/1 -> din1_0/1, din1_2/1
  din0_1/1 -> din1_1/1, din1_3/1
  din1_0/1 -> bussify/1(in1)
  din1_1/1 -> bussify/2(in2)
  din1_2/1 -> bussify/3(in3)
  din1_3/1 -> bussify/4(in4)
  bussify/1(bus_out) -> out/1

== system pfb_fft_d3a/fft_wideband_real/fft_biplex_real_4x/bi_real_unscr_4x/reorder_out/buf0 ==
  addr : Inport
  din : Inport  Port=2
  we : Inport  Port=3
  bram{0..3} (4 alike) : xbsIndex_r4/Single Port RAM  depth=1024  initVector=getfield(get_param(gcb, 'UserData'), 'initVector')  distributed_mem=Block RAM  write_mode=Read Before Write  rst=off  init_reg=0  en=off  optimize_latency=off  latency=2  optimize=Speed  dbl_ovrd=off  simulation_type=fast_sim  block_type=spram
  ddin : xbsIndex_r4/Delay  rst=off  infoeditControl=Selection of Reset will increase slice count due to use of real FFs and instead of SRLs  en=off  latency=3  reg_retiming=on  dbl_ovrd=off  block_type=delay
  debus_addr : Subsystem  AncestorBlock=casper_library_flow_control/bus_expand  mask(bus_expand){mode=divisions of equal size, outputNum=4, outputWidth=[10 10 10 10], outputBinaryPt=[0 0 0 0], outputArithmeticType=[0 0 0 0], show_format=on, outputToWorkspace=off, variablePrefix=, outputToModelAsWell=on}
      mask prompts: outputNum "Number of outputs:"; outputWidth "Output width:"; outputBinaryPt "Output binary point position:"; outputArithmeticType "Output arithmetic type (ufix=0, fix=1, bool=2):"; show_format "Print format string?"; outputToWorkspace "Output to workspace?"; variablePrefix "Variable name prefix:"; outputToModelAsWell "Output to model as well?"
      mask help:
      | Expands a 'bus' made using a bus_create or Xilinx
      | concat block.
      | The input will be divided into the specified number
      | of outputs with the specified arithmetic types.
      | Divisions are made from most significant bit.
      mask init: same as pfb_fft_d3a/fft_wideband_real/fft_biplex_real_4x/pol0_debus
      settings: AttributesFormatString=4 outputs: uf10.0,uf10.0,uf10.0,uf10.0,
      mask TypeOptions mode: divisions of equal size | divisions of arbitrary size
      mask Callback mode: %bus_expand_callback();
      mask Callback outputWidth: %bus_expand_callback();
      mask Callback outputToWorkspace: %bus_expand_callback();
  debus_din : Subsystem  AncestorBlock=casper_library_flow_control/bus_expand  mask(bus_expand){mode=divisions of arbitrary size, outputNum=2, outputWidth=[18 18 18 18], outputBinaryPt=[0 0 0 0], outputArithmeticType=[0 0 0 0], show_format=on, outputToWorkspace=off, variablePrefix=, outputToModelAsWell=on}
      mask prompts: outputNum "Number of outputs:"; outputWidth "Output width:"; outputBinaryPt "Output binary point position:"; outputArithmeticType "Output arithmetic type (ufix=0, fix=1, bool=2):"; show_format "Print format string?"; outputToWorkspace "Output to workspace?"; variablePrefix "Variable name prefix:"; outputToModelAsWell "Output to model as well?"
      mask help:
      | Expands a 'bus' made using a bus_create or Xilinx
      | concat block.
      | The input will be divided into the specified number
      | of outputs with the specified arithmetic types.
      | Divisions are made from most significant bit.
      mask init: same as pfb_fft_d3a/fft_wideband_real/fft_biplex_real_4x/pol0_debus
      settings: AttributesFormatString=4 outputs: uf18.0,uf18.0,uf18.0,uf18.0,
      mask TypeOptions mode: divisions of equal size | divisions of arbitrary size
      mask Callback mode: %bus_expand_callback();
      mask Callback outputWidth: %bus_expand_callback();
      mask Callback outputToWorkspace: %bus_expand_callback();
  debus_we : Subsystem  AncestorBlock=casper_library_flow_control/bus_expand  mask(bus_expand){mode=divisions of equal size, outputNum=4, outputWidth=[1 1 1 1], outputBinaryPt=[0 0 0 0], outputArithmeticType=[2 2 2 2], show_format=on, outputToWorkspace=off, variablePrefix=, outputToModelAsWell=on}
      mask prompts: outputNum "Number of outputs:"; outputWidth "Output width:"; outputBinaryPt "Output binary point position:"; outputArithmeticType "Output arithmetic type (ufix=0, fix=1, bool=2):"; show_format "Print format string?"; outputToWorkspace "Output to workspace?"; variablePrefix "Variable name prefix:"; outputToModelAsWell "Output to model as well?"
      mask help:
      | Expands a 'bus' made using a bus_create or Xilinx
      | concat block.
      | The input will be divided into the specified number
      | of outputs with the specified arithmetic types.
      | Divisions are made from most significant bit.
      mask init: same as pfb_fft_d3a/fft_wideband_real/fft_biplex_real_4x/pol0_debus
      settings: AttributesFormatString=4 outputs: b,b,b,b,
      mask TypeOptions mode: divisions of equal size | divisions of arbitrary size
      mask Callback mode: %bus_expand_callback();
      mask Callback outputWidth: %bus_expand_callback();
      mask Callback outputToWorkspace: %bus_expand_callback();
  din_bussify : Subsystem  AncestorBlock=casper_library_flow_control/bus_create  mask(bus_create){inputNum=4}
      mask prompts: inputNum "Number of inputs:"
      mask init:
      | bus_create_init(gcb,...
      |     'inputNum', inputNum);
  rep_addr : Subsystem  AncestorBlock=casper_library_bus/bus_replicate  mask(bus_replicate){replication=4, csp_latency=3, misc=off, implementation=core}
      mask prompts: replication "replication factor"; csp_latency "latency"; misc "misc support"; implementation "delay implementation"
      mask help: Output bus formed by replicating input bus a number of times
      mask init:
      | bus_replicate_init(gcb, ...
      |     'replication', replication, ...
      |     'csp_latency', csp_latency, ...
      |     'implementation', implementation, ...
      |     'misc', misc);
      mask TypeOptions implementation: core | behavioral
  rep_we : Subsystem  AncestorBlock=casper_library_bus/bus_replicate  mask(bus_replicate){replication=4, csp_latency=3, misc=off, implementation=core}
      mask prompts: replication "replication factor"; csp_latency "latency"; misc "misc support"; implementation "delay implementation"
      mask help: Output bus formed by replicating input bus a number of times
      mask init:
      | bus_replicate_init(gcb, ...
      |     'replication', replication, ...
      |     'csp_latency', csp_latency, ...
      |     'implementation', implementation, ...
      |     'misc', misc);
      mask TypeOptions implementation: core | behavioral
  dout : Outport
  wires:
  addr/1 -> rep_addr/1(in)
  din/1 -> ddin/1
  we/1 -> rep_we/1(in)
  rep_addr/1(out) -> debus_addr/1(bus_in)
  ddin/1 -> debus_din/1(bus_in)
  rep_we/1(out) -> debus_we/1(bus_in)
  debus_addr/1(msb_out4) -> bram0/1
  debus_din/1(msb_out4) -> bram0/2
  debus_we/1(msb_out4) -> bram0/3
  debus_addr/2(out3) -> bram1/1
  debus_din/2(out3) -> bram1/2
  debus_we/2(out3) -> bram1/3
  debus_addr/3(out2) -> bram2/1
  debus_din/3(out2) -> bram2/2
  debus_we/3(out2) -> bram2/3
  debus_addr/4(lsb_out1) -> bram3/1
  debus_din/4(lsb_out1) -> bram3/2
  debus_we/4(lsb_out1) -> bram3/3
  bram0/1 -> din_bussify/1(in1)
  bram1/1 -> din_bussify/2(in2)
  bram2/1 -> din_bussify/3(in3)
  bram3/1 -> din_bussify/4(in4)
  din_bussify/1(bus_out) -> dout/1

== system pfb_fft_d3a/fft_wideband_real/fft_biplex_real_4x/bi_real_unscr_4x/reorder_out/buf1 ==
  addr : Inport
  din : Inport  Port=2
  we : Inport  Port=3
  bram{0..3} (4 alike) : xbsIndex_r4/Single Port RAM  depth=1024  initVector=getfield(get_param(gcb, 'UserData'), 'initVector')  distributed_mem=Block RAM  write_mode=Read Before Write  rst=off  init_reg=0  en=off  optimize_latency=off  latency=2  optimize=Speed  dbl_ovrd=off  simulation_type=fast_sim  block_type=spram
  ddin : xbsIndex_r4/Delay  rst=off  infoeditControl=Selection of Reset will increase slice count due to use of real FFs and instead of SRLs  en=off  latency=3  reg_retiming=on  dbl_ovrd=off  block_type=delay
  debus_addr : Subsystem  AncestorBlock=casper_library_flow_control/bus_expand  mask(bus_expand){mode=divisions of equal size, outputNum=4, outputWidth=[10 10 10 10], outputBinaryPt=[0 0 0 0], outputArithmeticType=[0 0 0 0], show_format=on, outputToWorkspace=off, variablePrefix=, outputToModelAsWell=on}
      mask prompts: outputNum "Number of outputs:"; outputWidth "Output width:"; outputBinaryPt "Output binary point position:"; outputArithmeticType "Output arithmetic type (ufix=0, fix=1, bool=2):"; show_format "Print format string?"; outputToWorkspace "Output to workspace?"; variablePrefix "Variable name prefix:"; outputToModelAsWell "Output to model as well?"
      mask help:
      | Expands a 'bus' made using a bus_create or Xilinx
      | concat block.
      | The input will be divided into the specified number
      | of outputs with the specified arithmetic types.
      | Divisions are made from most significant bit.
      mask init: same as pfb_fft_d3a/fft_wideband_real/fft_biplex_real_4x/pol0_debus
      settings: AttributesFormatString=4 outputs: uf10.0,uf10.0,uf10.0,uf10.0,
      mask TypeOptions mode: divisions of equal size | divisions of arbitrary size
      mask Callback mode: %bus_expand_callback();
      mask Callback outputWidth: %bus_expand_callback();
      mask Callback outputToWorkspace: %bus_expand_callback();
  debus_din : Subsystem  AncestorBlock=casper_library_flow_control/bus_expand  mask(bus_expand){mode=divisions of arbitrary size, outputNum=2, outputWidth=[18 18 18 18], outputBinaryPt=[0 0 0 0], outputArithmeticType=[0 0 0 0], show_format=on, outputToWorkspace=off, variablePrefix=, outputToModelAsWell=on}
      mask prompts: outputNum "Number of outputs:"; outputWidth "Output width:"; outputBinaryPt "Output binary point position:"; outputArithmeticType "Output arithmetic type (ufix=0, fix=1, bool=2):"; show_format "Print format string?"; outputToWorkspace "Output to workspace?"; variablePrefix "Variable name prefix:"; outputToModelAsWell "Output to model as well?"
      mask help:
      | Expands a 'bus' made using a bus_create or Xilinx
      | concat block.
      | The input will be divided into the specified number
      | of outputs with the specified arithmetic types.
      | Divisions are made from most significant bit.
      mask init: same as pfb_fft_d3a/fft_wideband_real/fft_biplex_real_4x/pol0_debus
      settings: AttributesFormatString=4 outputs: uf18.0,uf18.0,uf18.0,uf18.0,
      mask TypeOptions mode: divisions of equal size | divisions of arbitrary size
      mask Callback mode: %bus_expand_callback();
      mask Callback outputWidth: %bus_expand_callback();
      mask Callback outputToWorkspace: %bus_expand_callback();
  debus_we : Subsystem  AncestorBlock=casper_library_flow_control/bus_expand  mask(bus_expand){mode=divisions of equal size, outputNum=4, outputWidth=[1 1 1 1], outputBinaryPt=[0 0 0 0], outputArithmeticType=[2 2 2 2], show_format=on, outputToWorkspace=off, variablePrefix=, outputToModelAsWell=on}
      mask prompts: outputNum "Number of outputs:"; outputWidth "Output width:"; outputBinaryPt "Output binary point position:"; outputArithmeticType "Output arithmetic type (ufix=0, fix=1, bool=2):"; show_format "Print format string?"; outputToWorkspace "Output to workspace?"; variablePrefix "Variable name prefix:"; outputToModelAsWell "Output to model as well?"
      mask help:
      | Expands a 'bus' made using a bus_create or Xilinx
      | concat block.
      | The input will be divided into the specified number
      | of outputs with the specified arithmetic types.
      | Divisions are made from most significant bit.
      mask init: same as pfb_fft_d3a/fft_wideband_real/fft_biplex_real_4x/pol0_debus
      settings: AttributesFormatString=4 outputs: b,b,b,b,
      mask TypeOptions mode: divisions of equal size | divisions of arbitrary size
      mask Callback mode: %bus_expand_callback();
      mask Callback outputWidth: %bus_expand_callback();
      mask Callback outputToWorkspace: %bus_expand_callback();
  din_bussify : Subsystem  AncestorBlock=casper_library_flow_control/bus_create  mask(bus_create){inputNum=4}
      mask prompts: inputNum "Number of inputs:"
      mask init:
      | bus_create_init(gcb,...
      |     'inputNum', inputNum);
  rep_addr : Subsystem  AncestorBlock=casper_library_bus/bus_replicate  mask(bus_replicate){replication=4, csp_latency=3, misc=off, implementation=core}
      mask prompts: replication "replication factor"; csp_latency "latency"; misc "misc support"; implementation "delay implementation"
      mask help: Output bus formed by replicating input bus a number of times
      mask init:
      | bus_replicate_init(gcb, ...
      |     'replication', replication, ...
      |     'csp_latency', csp_latency, ...
      |     'implementation', implementation, ...
      |     'misc', misc);
      mask TypeOptions implementation: core | behavioral
  rep_we : Subsystem  AncestorBlock=casper_library_bus/bus_replicate  mask(bus_replicate){replication=4, csp_latency=3, misc=off, implementation=core}
      mask prompts: replication "replication factor"; csp_latency "latency"; misc "misc support"; implementation "delay implementation"
      mask help: Output bus formed by replicating input bus a number of times
      mask init:
      | bus_replicate_init(gcb, ...
      |     'replication', replication, ...
      |     'csp_latency', csp_latency, ...
      |     'implementation', implementation, ...
      |     'misc', misc);
      mask TypeOptions implementation: core | behavioral
  dout : Outport
  wires:
  addr/1 -> rep_addr/1(in)
  din/1 -> ddin/1
  we/1 -> rep_we/1(in)
  rep_addr/1(out) -> debus_addr/1(bus_in)
  ddin/1 -> debus_din/1(bus_in)
  rep_we/1(out) -> debus_we/1(bus_in)
  debus_addr/1(msb_out4) -> bram0/1
  debus_din/1(msb_out4) -> bram0/2
  debus_we/1(msb_out4) -> bram0/3
  debus_addr/2(out3) -> bram1/1
  debus_din/2(out3) -> bram1/2
  debus_we/2(out3) -> bram1/3
  debus_addr/3(out2) -> bram2/1
  debus_din/3(out2) -> bram2/2
  debus_we/3(out2) -> bram2/3
  debus_addr/4(lsb_out1) -> bram3/1
  debus_din/4(lsb_out1) -> bram3/2
  debus_we/4(lsb_out1) -> bram3/3
  bram0/1 -> din_bussify/1(in1)
  bram1/1 -> din_bussify/2(in2)
  bram2/1 -> din_bussify/3(in3)
  bram3/1 -> din_bussify/4(in4)
  din_bussify/1(bus_out) -> dout/1
